simulink subsystem "navigationcopycopy"  (R2026a)
settings: Solver=VariableStepAuto
values from neighbouring files (symbols this model uses):
  navComp = 0.99    [navParams.sldd]
  navControl = 1    [navParams.sldd]
undefined symbols (not defined in the file or in its folder): flightMode
libraries: sharedutil x2, simulink x2, aerolibutil x1, matrix_library x1
settings Model: DataDictionary=navParams.sldd  EnableAccessToBaseWorkspace=off  Creator=maxhu  LastModifiedBy=nathanscott

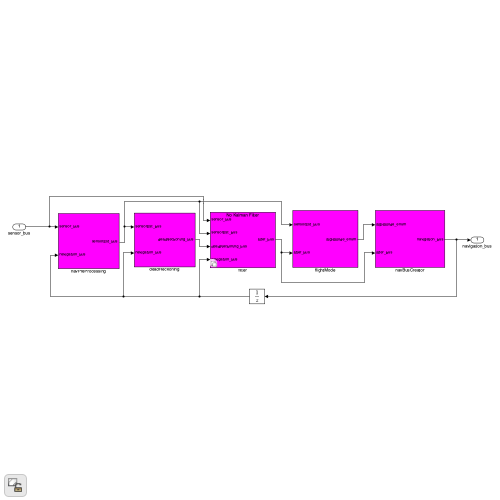
[thumbnail: Simulink's stored preview of the top-level diagram]
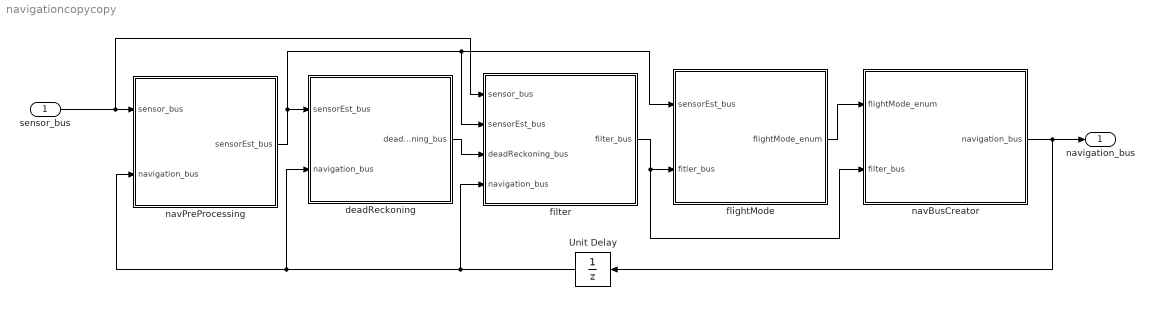
== system navigationcopycopy ==
  sensor_bus : Inport
  Unit Delay : UnitDelay  SampleTime=navControl.dt_s
  deadReckoning : Subsystem
  filter : Subsystem  Variant=on
  flightMode : Subsystem
  navBusCreator : Subsystem
  navPreProcessing : Subsystem
  navigation_bus : Outport
  wires:
  navBusCreator/1(navigation_bus) -> navigation_bus/1, Unit Delay/1
  flightMode/1(flightMode_enum) -> navBusCreator/1(flightMode_enum)
  sensor_bus/1 -> navPreProcessing/1(sensor_bus), filter/1(sensor_bus)
  navPreProcessing/1(sensorEst_bus) -> filter/2(sensorEst_bus), flightMode/1(sensorEst_bus), deadReckoning/1(sensorEst_bus)
  deadReckoning/1(deadReckoning_bus) -> filter/3(deadReckoning_bus)
  filter/1(filter_bus) -> navBusCreator/2(filter_bus), flightMode/2(fitler_bus)
  Unit Delay/1 -> deadReckoning/2(navigation_bus), navPreProcessing/2(navigation_bus), filter/4(navigation_bus)

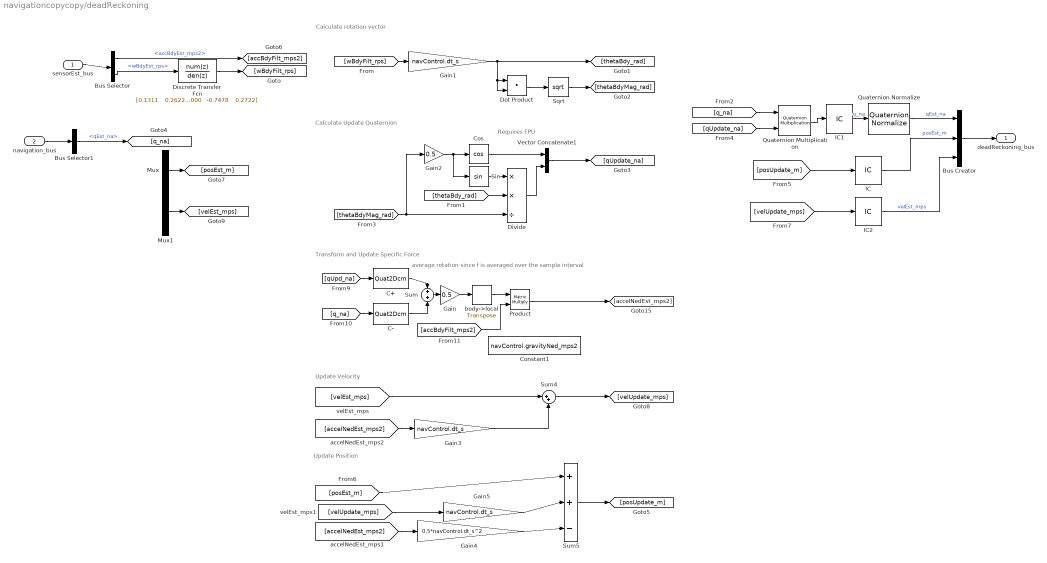
== system navigationcopycopy/deadReckoning ==
  note: Update Velocity
  note: Transform and Update
      |  Specific Force
  note: average rotation since f is averaged over the sample interval
  note: Update Position
  note: Requires FPU
  note: Calculate rotation vector
  note: Calculate Update Quaternion
  sensorEst_bus : Inport
  navigation_bus : Inport  Port=2
  Bus Creator : BusCreator  Inputs=3
  Bus Selector : BusSelector  OutputSignals=accBdyEst_mps2,wBdyEst_rps
  Bus Selector1 : BusSelector  OutputSignals=qEst_na
  C+ : Quat2Dcm
  C- : Quat2Dcm
  Constant1 : Constant  Value=navControl.gravityNed_mps2
  Cos : Trigonometry  Operator=cos
  Discrete Transfer Fcn : DiscreteTransferFcn  Numerator="[0.1311    0.2622    0.1311]"  Denominator="[1.0000   -0.7478    0.2722]"
  Divide : Product  Inputs=**/
  Dot Product : DotProduct  OutDataTypeStr=Inherit: Inherit via internal rule
  Gain : Gain  Gain=0.5
  Gain1 : Gain  Gain=navControl.dt_s
  Gain2 : Gain  Gain=0.5
  Gain3 : Gain  Gain=navControl.dt_s
  Gain4 : Gain  Gain=0.5*navControl.dt_s^2
  Gain5 : Gain  Gain=navControl.dt_s
  IC : InitialCondition  Value=navControl.posNed0_m
  IC1 : InitialCondition  Value=navControl.q0_na
  IC2 : InitialCondition  Value=navControl.velNed0_mps
  Mux : Mux  Inputs=3
  Mux1 : Mux  Inputs=3
  Product : Product  Multiplication=Matrix(*)
  Quaternion Multiplication : aerolibutil/Quaternion Multiplication
  Quaternion Normalize : sharedutil/Quaternion Normalize  aMode=aMode
  Sin : Trigonometry
  Sqrt : Sqrt
  Sum : Sum  Inputs=+|+
  Sum4 : Sum  Inputs=|++
  Sum5 : Sum  Inputs=|++-
  Vector Concatenate1 : Concatenate
  body->local : matrix_library/Transpose
  deadReckoning_bus : Outport
  wires:
  ? -> Mux/1  "<xPosEst_m>"
  ? -> Mux1/1  "<xVelEst_mps>"
  Mux1/1 -> [velEst_mps]
  ? -> Mux/2  "<yPosEst_m>"
  ? -> Mux1/2  "<yVelEst_mps>"
  ? -> Mux1/3  "<zVelEst_mps>"
  ? -> Mux/3  "<zPosEst_m>"
  Mux/1 -> [posEst_m]
  Gain3/1 -> Sum4/2
  Bus Selector/1 -> [accBdyFilt_mps2]  "<accBdyEst_mps2>"
  IC2/1 -> Bus Creator/3  "velEst_mps"
  IC/1 -> Bus Creator/2  "posEst_m"
  [velUpdate_mps] -> IC2/1
  [posUpdate_m] -> IC/1
  [q_na] -> C-/1
  Gain4/1 -> Sum5/3
  Gain/1 -> body->local/1
  [qUpd_na] -> C+/1
  C-/1 -> Sum/2
  [accBdyFilt_mps2] -> Product/2
  [accelNedEst_mps2] -> Gain3/1
  Product/1 -> [accelNedEst_mps2]
  Sum5/1 -> [posUpdate_m]
  body->local/1 -> Product/1
  [accelNedEst_mps2] -> Gain4/1
  Gain5/1 -> Sum5/2
  Sum/1 -> Gain/1
  [posEst_m] -> Sum5/1
  [velEst_mps] -> Sum4/1
  Sum4/1 -> [velUpdate_mps]
  [velUpdate_mps] -> Gain5/1
  C+/1 -> Sum/1
  Bus Creator/1 -> deadReckoning_bus/1
  IC1/1 -> Quaternion Normalize/1  "q_na"
  Quaternion Normalize/1 -> Bus Creator/1  "qEst_na"
  Discrete Transfer Fcn/1 -> [wBdyFilt_rps]
  Bus Selector/2 -> Discrete Transfer Fcn/1  "<wBdyEst_rps>"
  Bus Selector1/1 -> [q_na]  "<qEst_na>"
  navigation_bus/1 -> Bus Selector1/1
  [thetaBdy_rad] -> Divide/2
  Quaternion Multiplication/1 -> IC1/1
  [qUpdate_na] -> Quaternion Multiplication/2
  [q_na] -> Quaternion Multiplication/1
  Vector Concatenate1/1 -> [qUpdate_na]
  Divide/1 -> Vector Concatenate1/2
  Cos/1 -> Vector Concatenate1/1
  Sin/1 -> Divide/1
  [thetaBdyMag_rad] -> Divide/3, Gain2/1
  Gain2/1 -> Cos/1, Sin/1
  Sqrt/1 -> [thetaBdyMag_rad]
  Gain1/1 -> [thetaBdy_rad], Dot Product/1, Dot Product/2
  Dot Product/1 -> Sqrt/1
  [wBdyFilt_rps] -> Gain1/1
  sensorEst_bus/1 -> Bus Selector/1

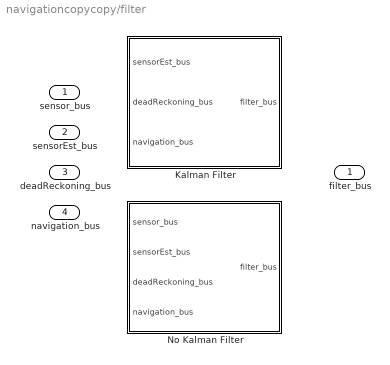
== system navigationcopycopy/filter ==
  sensor_bus : Inport
  sensorEst_bus : Inport  Port=2
  deadReckoning_bus : Inport  Port=3
  navigation_bus : Inport  Port=4
  Kalman Filter : Subsystem  VariantControl=navControl.useKalman_b == true
  No Kalman Filter : Subsystem  VariantControl=navControl.useKalman_b == false
  filter_bus : Outport

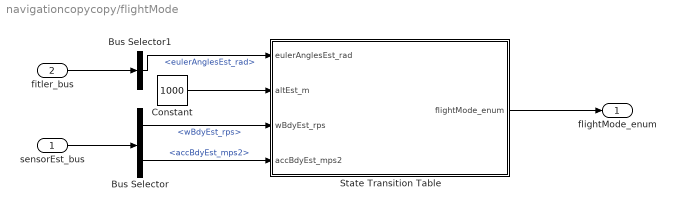
== system navigationcopycopy/flightMode ==
  sensorEst_bus : Inport
  fitler_bus : Inport  Port=2
  Bus Selector : BusSelector  OutputSignals=wBdyEst_rps,accBdyEst_mps2
  Bus Selector1 : BusSelector  OutputSignals=eulerAnglesEst_rad
  Constant : Constant  Value=1000
  State Transition Table : State Transition Table  TreatAsAtomicUnit=on
  flightMode_enum : Outport
  wires:
  fitler_bus/1 -> Bus Selector1/1
  Bus Selector1/1 -> State Transition Table/1(eulerAnglesEst_rad)  "<eulerAnglesEst_rad>"
  Constant/1 -> State Transition Table/2(altEst_m)
  State Transition Table/1(flightMode_enum) -> flightMode_enum/1
  Bus Selector/1 -> State Transition Table/3(wBdyEst_rps)  "<wBdyEst_rps>"
  Bus Selector/2 -> State Transition Table/4(accBdyEst_mps2)  "<accBdyEst_mps2>"
  sensorEst_bus/1 -> Bus Selector/1

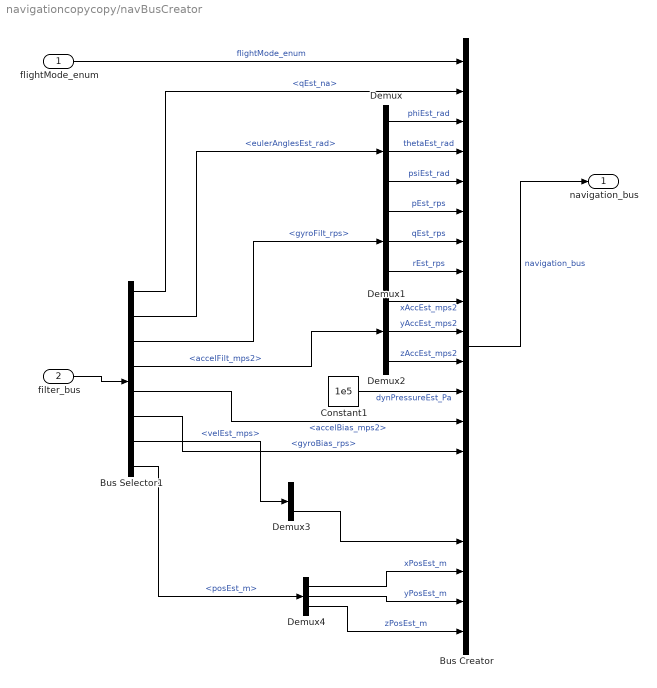
== system navigationcopycopy/navBusCreator ==
  flightMode_enum : Inport
  filter_bus : Inport  Port=2
  Bus Creator : BusCreator  Inputs=20
  Bus Selector1 : BusSelector  OutputSignals=qEst_na,eulerAnglesEst_rad,gyroFilt_rps,accelFilt_mps2,accelBias_mps2,gyroBias_rps,velEst_mps,posEst_m
  Constant1 : Constant  Value=1e5
  Demux{,1..2,4} (4 alike) : Demux  Outputs=3
  Demux3 : Demux  Outputs=2
  navigation_bus : Outport
  wires:
  Demux4/3 -> Bus Creator/20  "zPosEst_m"
  Demux4/2 -> Bus Creator/19  "yPosEst_m"
  Demux4/1 -> Bus Creator/18  "xPosEst_m"
  Bus Selector1/8 -> Demux4/1  "<posEst_m>"
  Bus Selector1/7 -> Demux3/1  "<velEst_mps>"
  Bus Selector1/4 -> Demux2/1  "<accelFilt_mps2>"
  Bus Selector1/3 -> Demux1/1  "<gyroFilt_rps>"
  Bus Selector1/6 -> Bus Creator/14  "<gyroBias_rps>"
  Bus Selector1/5 -> Bus Creator/13  "<accelBias_mps2>"
  Demux2/3 -> Bus Creator/11  "zAccEst_mps2"
  Demux2/2 -> Bus Creator/10  "yAccEst_mps2"
  Demux2/1 -> Bus Creator/9  "xAccEst_mps2"
  Bus Selector1/1 -> Bus Creator/2  "<qEst_na>"
  filter_bus/1 -> Bus Selector1/1
  flightMode_enum/1 -> Bus Creator/1  "flightMode_enum"
  Bus Selector1/2 -> Demux/1  "<eulerAnglesEst_rad>"
  Bus Creator/1 -> navigation_bus/1  "navigation_bus"
  Demux1/2 -> Bus Creator/7  "qEst_rps"
  Constant1/1 -> Bus Creator/12  "dynPressureEst_Pa"
  Demux1/1 -> Bus Creator/6  "pEst_rps"
  Demux/3 -> Bus Creator/5  "psiEst_rad"
  Demux1/3 -> Bus Creator/8  "rEst_rps"
  Demux/1 -> Bus Creator/3  "phiEst_rad"
  Demux/2 -> Bus Creator/4  "thetaEst_rad"
  Demux3/2 -> Bus Creator/17

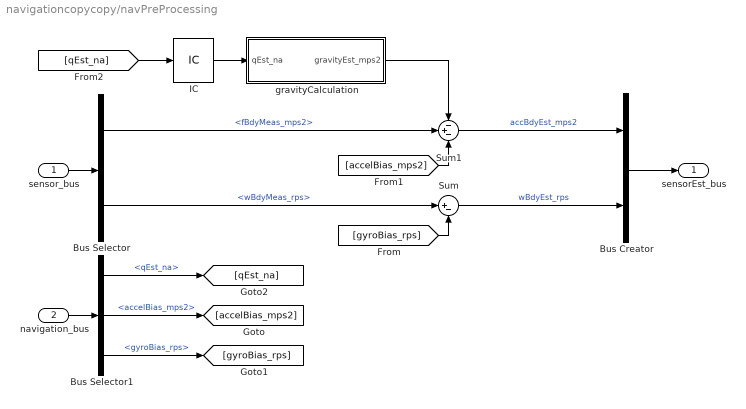
== system navigationcopycopy/navPreProcessing ==
  sensor_bus : Inport
  navigation_bus : Inport  Port=2
  Bus Creator : BusCreator  Inputs=2
  Bus Selector : BusSelector  OutputSignals=fBdyMeas_mps2,wBdyMeas_rps
  Bus Selector1 : BusSelector  OutputSignals=qEst_na,accelBias_mps2,gyroBias_rps
  IC : InitialCondition  Value=[1,0,0,0]
  Sum : Sum  Inputs=|+-
  Sum1 : Sum  Inputs=-+-
  gravityCalculation : Subsystem
  sensorEst_bus : Outport
  wires:
  gravityCalculation/1(gravityEst_mps2) -> Sum1/1
  [accelBias_mps2] -> Sum1/3
  [gyroBias_rps] -> Sum/2
  IC/1 -> gravityCalculation/1(qEst_na)
  [qEst_na] -> IC/1
  Bus Selector/1 -> Sum1/2  "<fBdyMeas_mps2>"
  Bus Selector1/1 -> [qEst_na]  "<qEst_na>"
  Bus Selector1/3 -> [gyroBias_rps]  "<gyroBias_rps>"
  Bus Selector1/2 -> [accelBias_mps2]  "<accelBias_mps2>"
  navigation_bus/1 -> Bus Selector1/1
  sensor_bus/1 -> Bus Selector/1
  Bus Selector/2 -> Sum/1  "<wBdyMeas_rps>"
  Bus Creator/1 -> sensorEst_bus/1
  Sum1/1 -> Bus Creator/1  "accBdyEst_mps2"
  Sum/1 -> Bus Creator/2  "wBdyEst_rps"

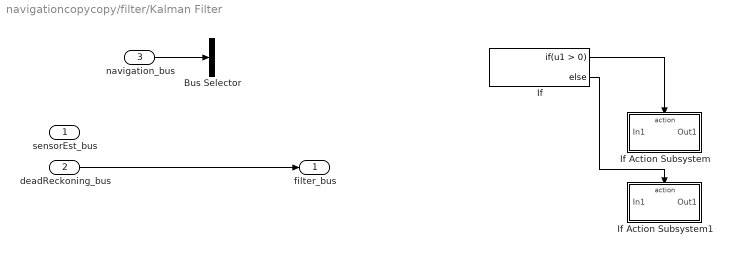
== system navigationcopycopy/filter/Kalman Filter ==
  sensorEst_bus : Inport
  deadReckoning_bus : Inport  Port=2
  navigation_bus : Inport  Port=3
  Bus Selector : BusSelector  OutputSignals=signal1,signal2
  If : If
  If Action Subsystem : Subsystem  TreatAsAtomicUnit=on
  If Action Subsystem1 : Subsystem  TreatAsAtomicUnit=on
  filter_bus : Outport
  wires:
  navigation_bus/1 -> Bus Selector/1
  If/2 -> If Action Subsystem1/Action
  If/1 -> If Action Subsystem/Action
  deadReckoning_bus/1 -> filter_bus/1

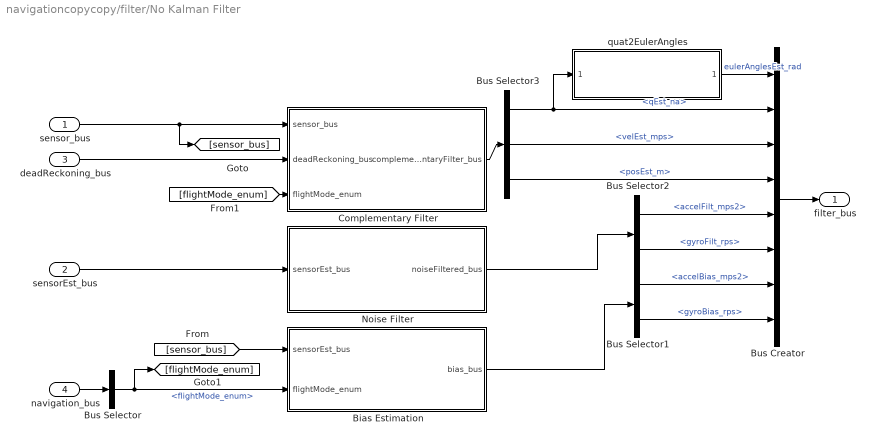
== system navigationcopycopy/filter/No Kalman Filter ==
  sensor_bus : Inport
  sensorEst_bus : Inport  Port=2
  deadReckoning_bus : Inport  Port=3
  navigation_bus : Inport  Port=4
  Bias Estimation : Subsystem
  Bus Creator : BusCreator  Inputs=8
  Bus Selector : BusSelector  OutputSignals=flightMode_enum
  Bus Selector1 : BusSelector  OutputSignals=accelBias_mps2,gyroBias_rps
  Bus Selector2 : BusSelector  OutputSignals=accelFilt_mps2,gyroFilt_rps
  Bus Selector3 : BusSelector  OutputSignals=qEst_na,velEst_mps,posEst_m
  Complementary Filter : Subsystem
  Noise Filter : Subsystem
  quat2EulerAngles : Subsystem  ReferencedSubsystem=quat2EulerAngles
  filter_bus : Outport
  wires:
  Bus Selector3/2 -> Bus Creator/3  "<velEst_mps>"
  Bus Selector3/3 -> Bus Creator/4  "<posEst_m>"
  deadReckoning_bus/1 -> Complementary Filter/2(deadReckoning_bus)
  [flightMode_enum] -> Complementary Filter/3(flightMode_enum)
  Complementary Filter/1(complementaryFilter_bus) -> Bus Selector3/1
  [sensor_bus] -> Bias Estimation/1(sensorEst_bus)
  Bus Creator/1 -> filter_bus/1
  Bus Selector2/1 -> Bus Creator/5  "<accelFilt_mps2>"
  quat2EulerAngles/1 -> Bus Creator/1  "eulerAnglesEst_rad"
  Bus Selector3/1 -> Bus Creator/2, quat2EulerAngles/1  "<qEst_na>"
  Bus Selector2/2 -> Bus Creator/6  "<gyroFilt_rps>"
  Bus Selector1/2 -> Bus Creator/8  "<gyroBias_rps>"
  Bus Selector1/1 -> Bus Creator/7  "<accelBias_mps2>"
  Bias Estimation/1(bias_bus) -> Bus Selector1/1
  sensor_bus/1 -> Complementary Filter/1(sensor_bus), [sensor_bus]
  Bus Selector/1 -> [flightMode_enum], Bias Estimation/2(flightMode_enum)  "<flightMode_enum>"
  Noise Filter/1(noiseFiltered_bus) -> Bus Selector2/1
  sensorEst_bus/1 -> Noise Filter/1(sensorEst_bus)
  navigation_bus/1 -> Bus Selector/1

== system navigationcopycopy/navPreProcessing/gravityCalculation ==
  qEst_na : Inport
  Constant : Constant  Value=navControl.gravityNed_mps2
  Matrix Multiply : Product  Multiplication=Matrix(*)
  Quaternions to Direction Cosine Matrix : Quat2Dcm
  gravityEst_mps2 : Outport
  wires:
  qEst_na/1 -> Quaternions to Direction Cosine Matrix/1
  Matrix Multiply/1 -> gravityEst_mps2/1
  Constant/1 -> Matrix Multiply/2
  Quaternions to Direction Cosine Matrix/1 -> Matrix Multiply/1

== system navigationcopycopy/filter/Kalman Filter/If Action Subsystem ==
  In1 : Inport
  Action Port : ActionPort
  Out1 : Outport
  wires:
  In1/1 -> Out1/1

== system navigationcopycopy/filter/Kalman Filter/If Action Subsystem1 ==
  In1 : Inport
  Action Port : ActionPort
  Out1 : Outport
  wires:
  In1/1 -> Out1/1

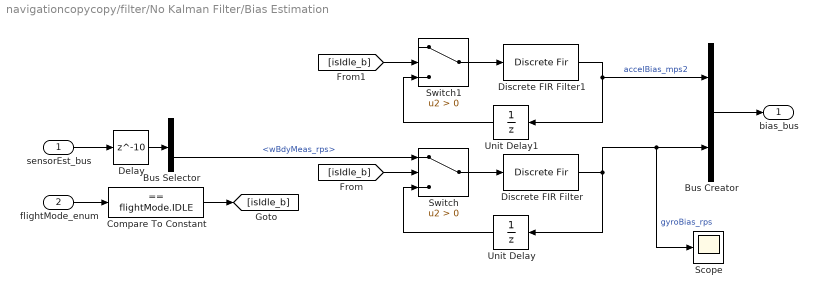
== system navigationcopycopy/filter/No Kalman Filter/Bias Estimation ==
  sensorEst_bus : Inport
  flightMode_enum : Inport  Port=2
  Bus Creator : BusCreator  Inputs=2
  Bus Selector : BusSelector  OutputSignals=fBdyMeas_mps2,wBdyMeas_rps
  Compare To Constant : simulink/Logic and Bit Operations/Compare To Constant  relop===  const=flightMode.IDLE  OutDataTypeStr=boolean
  Delay : Delay  DelayLength=10
  Discrete FIR Filter : DiscreteFir  Coefficients=ones(1,100)/100
  Discrete FIR Filter1 : DiscreteFir  Coefficients=ones(1,100)/100
  Scope : Scope
      settings: ActiveDisplayYMinimum=-0.019193528389318905  ActiveDisplayYMaximum=-0.01541623972070829
  Switch : Switch  Criteria=u2 > Threshold  SaturateOnIntegerOverflow=off  InputSameDT=off
  Switch1 : Switch  Criteria=u2 > Threshold  SaturateOnIntegerOverflow=off  InputSameDT=off
  Unit Delay : UnitDelay  SampleTime=-1
  Unit Delay1 : UnitDelay  SampleTime=-1
  bias_bus : Outport
  wires:
  Bus Creator/1 -> bias_bus/1
  Discrete FIR Filter1/1 -> Bus Creator/1, Unit Delay1/1  "accelBias_mps2"
  [isIdle_b] -> Switch1/2
  Switch1/1 -> Discrete FIR Filter1/1
  Unit Delay1/1 -> Switch1/3
  Delay/1 -> Bus Selector/1
  [isIdle_b] -> Switch/2
  Compare To Constant/1 -> [isIdle_b]
  Bus Selector/2 -> Switch/1  "<wBdyMeas_rps>"
  sensorEst_bus/1 -> Delay/1
  flightMode_enum/1 -> Compare To Constant/1
  Switch/1 -> Discrete FIR Filter/1
  Unit Delay/1 -> Switch/3
  Discrete FIR Filter/1 -> Bus Creator/2, Scope/1, Unit Delay/1  "gyroBias_rps"

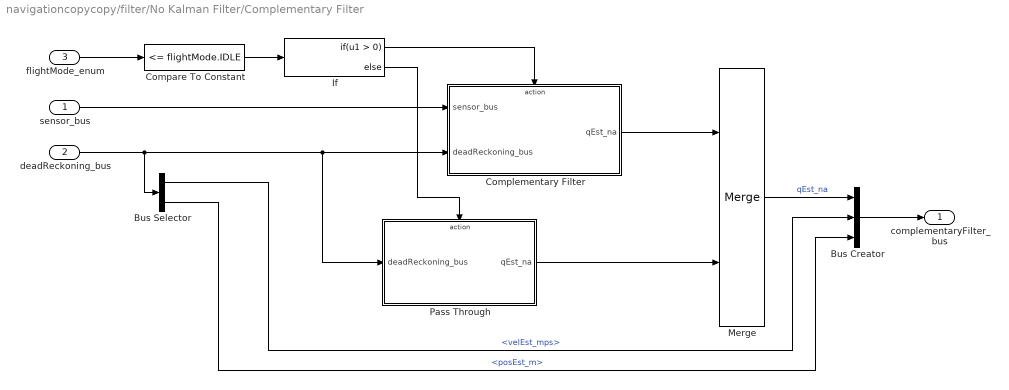
== system navigationcopycopy/filter/No Kalman Filter/Complementary Filter ==
  sensor_bus : Inport
  deadReckoning_bus : Inport  Port=2
  flightMode_enum : Inport  Port=3
  Bus Creator : BusCreator  Inputs=3
  Bus Selector : BusSelector  OutputSignals=velEst_mps,posEst_m
  Compare To Constant : simulink/Logic and Bit Operations/Compare To Constant  relop=<=  const=flightMode.IDLE  OutDataTypeStr=boolean
  Complementary Filter : Subsystem  TreatAsAtomicUnit=on
  If : If
  Merge : Merge
  Pass Through : Subsystem  TreatAsAtomicUnit=on
  complementaryFilter_bus : Outport
  wires:
  Bus Selector/2 -> Bus Creator/3  "<posEst_m>"
  Bus Selector/1 -> Bus Creator/2  "<velEst_mps>"
  Pass Through/1(qEst_na) -> Merge/2
  Complementary Filter/1(qEst_na) -> Merge/1
  sensor_bus/1 -> Complementary Filter/1(sensor_bus)
  deadReckoning_bus/1 -> Complementary Filter/2(deadReckoning_bus), Pass Through/1(deadReckoning_bus), Bus Selector/1
  If/2 -> Pass Through/Action
  If/1 -> Complementary Filter/Action
  Compare To Constant/1 -> If/1
  flightMode_enum/1 -> Compare To Constant/1
  Bus Creator/1 -> complementaryFilter_bus/1
  Merge/1 -> Bus Creator/1  "qEst_na"

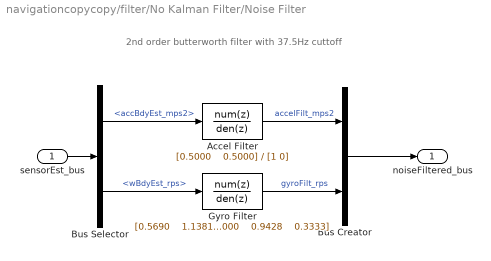
== system navigationcopycopy/filter/No Kalman Filter/Noise Filter ==
  note: 2nd order butterworth filter with 37.5Hz cuttoff
  sensorEst_bus : Inport
  Accel Filter : DiscreteTransferFcn  Numerator="[0.5000    0.5000]"  Denominator=[1 0]
  Bus Creator : BusCreator  Inputs=2
  Bus Selector : BusSelector  OutputSignals=accBdyEst_mps2,wBdyEst_rps
  Gyro Filter : DiscreteTransferFcn  Numerator="[0.5690    1.1381    0.5690]"  Denominator="[1.0000    0.9428    0.3333]"
  noiseFiltered_bus : Outport
  wires:
  Bus Selector/1 -> Accel Filter/1  "<accBdyEst_mps2>"
  Accel Filter/1 -> Bus Creator/1  "accelFilt_mps2"
  Gyro Filter/1 -> Bus Creator/2  "gyroFilt_rps"
  Bus Selector/2 -> Gyro Filter/1  "<wBdyEst_rps>"
  Bus Creator/1 -> noiseFiltered_bus/1
  sensorEst_bus/1 -> Bus Selector/1

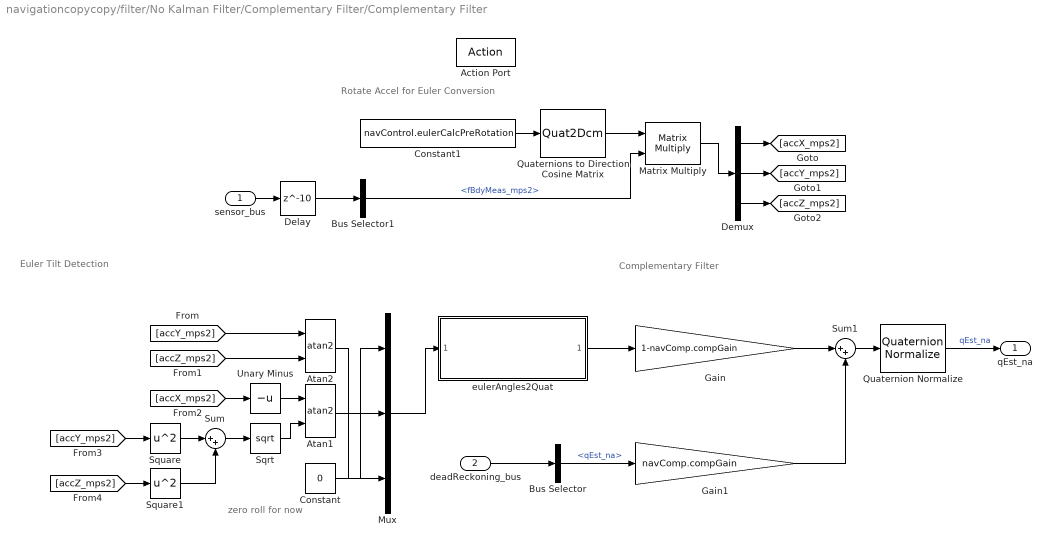
== system navigationcopycopy/filter/No Kalman Filter/Complementary Filter/Complementary Filter ==
  note: Rotate Accel for Euler Conversion
  note: Euler Tilt Detection
  note: Complementary Filter
  note: zero roll for now
  sensor_bus : Inport
  deadReckoning_bus : Inport  Port=2
  Action Port : ActionPort
  Atan1 : Trigonometry  Operator=atan2
  Atan2 : Trigonometry  Operator=atan2
  Bus Selector : BusSelector  OutputSignals=qEst_na
  Bus Selector1 : BusSelector  OutputSignals=fBdyMeas_mps2
  Constant : Constant  Value=0
  Constant1 : Constant  Value=navControl.eulerCalcPreRotation
  Delay : Delay  DelayLength=10
  Demux : Demux  Outputs=3
  Gain : Gain  Gain=1-navComp.compGain
  Gain1 : Gain  Gain=navComp.compGain
  Matrix Multiply : Product  Multiplication=Matrix(*)
  Mux : Mux  Inputs=3
  Quaternion Normalize : sharedutil/Quaternion Normalize  aMode=aMode
  Quaternions to Direction Cosine Matrix : Quat2Dcm
  Sqrt : Sqrt
  Square : Math  Operator=square
  Square1 : Math  Operator=square
  Sum : Sum  Inputs=|++
  Sum1 : Sum  Inputs=|++
  Unary Minus : UnaryMinus
  eulerAngles2Quat : Subsystem  ReferencedSubsystem=eulerAngles2Quat
  qEst_na : Outport
  wires:
  Atan2/1 -> Mux/3
  Constant/1 -> Mux/1
  Quaternion Normalize/1 -> qEst_na/1  "qEst_na"
  Matrix Multiply/1 -> Demux/1
  [accY_mps2] -> Square/1
  Gain1/1 -> Sum1/2
  Bus Selector/1 -> Gain1/1  "<qEst_na>"
  Square/1 -> Sum/1
  Sum/1 -> Sqrt/1
  Atan1/1 -> Mux/2
  eulerAngles2Quat/1 -> Gain/1
  Demux/1 -> [accX_mps2]
  sensor_bus/1 -> Delay/1
  Bus Selector1/1 -> Matrix Multiply/2  "<fBdyMeas_mps2>"
  Square1/1 -> Sum/2
  Gain/1 -> Sum1/1
  Demux/2 -> [accY_mps2]
  Demux/3 -> [accZ_mps2]
  Unary Minus/1 -> Atan1/1
  [accZ_mps2] -> Square1/1
  Sum1/1 -> Quaternion Normalize/1
  Sqrt/1 -> Atan1/2
  Constant1/1 -> Quaternions to Direction Cosine Matrix/1
  deadReckoning_bus/1 -> Bus Selector/1
  Mux/1 -> eulerAngles2Quat/1
  Delay/1 -> Bus Selector1/1
  [accY_mps2] -> Atan2/1
  [accX_mps2] -> Unary Minus/1
  [accZ_mps2] -> Atan2/2
  Quaternions to Direction Cosine Matrix/1 -> Matrix Multiply/1

== system navigationcopycopy/filter/No Kalman Filter/Complementary Filter/Pass Through ==
  deadReckoning_bus : Inport
  Action Port : ActionPort
  Bus Selector : BusSelector  OutputSignals=qEst_na
  qEst_na : Outport
  wires:
  Bus Selector/1 -> qEst_na/1  "<qEst_na>"
  deadReckoning_bus/1 -> Bus Selector/1

== stateflow chart navigationcopycopy/flightMode/State Transition Table ==
  state Idle
    entry:
    flightMode_enum = flightMode.IDLE;
    boostThreshold_b = false;
    during:
    boostThreshold_b = norm(accBdyEst_mps2) > navStates.boostThreshold_mps2;
  state Boost
    entry:
    flightMode_enum = flightMode.BOOST;
    coastThreshold_b = false;
    during:
    coastThreshold_b = altEst_m > navStates.coastThresholdAlt_m && ...
    accBdyEst_mps2(1) < navStates.coastThresholdxAcc_mps2;
  state PastCoastThreshold
    during:
    coastThreshold_b = altEst_m > navStates.coastThresholdAlt_m && ...
    accBdyEst_mps2(1) < navStates.coastThresholdxAcc_mps2;
  state Active
    entry:
    flightMode_enum = flightMode.ACTIVE;
    lockoutThreshold_b = false;
    during:
    lockoutThreshold_b = wBdyEst_rps(2) > navStates.controlTresholdPitchYawRate_rps || ...
    wBdyEst_rps(3) > navStates.controlTresholdPitchYawRate_rps || ...
    eulerAnglesEst_rad(2) > navStates.controlTresholdPitchYaw_rad || ...
    eulerAnglesEst_rad(3) > navStates.controlTresholdPitchYaw_rad;
  state PastLockoutThreshold
    during:
    lockoutThreshold_b = wBdyEst_rps(2) > navStates.controlTresholdPitchYawRate_rps || ...
    wBdyEst_rps(3) > navStates.controlTresholdPitchYawRate_rps || ...
    eulerAnglesEst_rad(2) > navStates.controlTresholdPitchYaw_rad || ...
    eulerAnglesEst_rad(3) > navStates.controlTresholdPitchYaw_rad;
  state Lockout
    entry:
    flightMode_enum = flightMode.LOCKOUT;
  (default) -> Idle
  Idle -> Boost : [boostThreshold_b]
  Boost -> PastCoastThreshold : [coastThreshold_b]
  PastCoastThreshold -> Boost [order 1] : [~coastThreshold_b]
  PastCoastThreshold -> Active [order 2] : [elapsed(sec) > navStates.debounce_s]
  Active -> PastLockoutThreshold : [lockoutThreshold_b]
  PastLockoutThreshold -> Active [order 1] : [~lockoutThreshold_b]
  PastLockoutThreshold -> Lockout [order 2] : [elapsed(sec) > navStates.debounce_s]
  data: eulerAnglesEst_rad input; boostThreshold_b local; lockoutThreshold_b local; flightMode_enum output; altEst_m input; coastThreshold_b local; wBdyEst_rps input; accBdyEst_mps2 input; navStates parameter
